simulink model "sfGetStartedBattery"  (R2025b)
settings: Solver=VariableStepAuto  StartTime=0.0  StopTime=inf  RelTol=1e-3
settings Model: Creator=The MathWorks, Inc.  LastModifiedBy=The MathWorks, Inc.

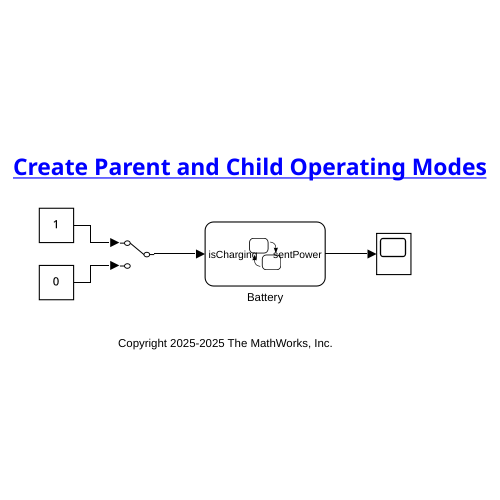
[thumbnail: Simulink's stored preview of the top-level diagram]
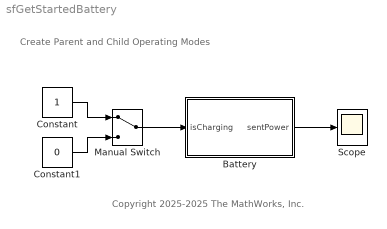
== system sfGetStartedBattery ==
  note: Copyright 2025-2025 The MathWorks, Inc.
  note: Create Parent and Child Operating Modes
  Battery : Stateflow chart  TreatAsAtomicUnit=on
  Constant : Constant
  Constant1 : Constant  Value=0
  Manual Switch : ManualSwitch
  Scope : Scope
      settings: ActiveDisplayYMinimum=-0.43749999999999989  ActiveDisplayYMaximum=3.9375
  wires:
  Manual Switch/1 -> Battery/1(isCharging)
  Constant/1 -> Manual Switch/1
  Constant1/1 -> Manual Switch/2
  Battery/1(sentPower) -> Scope/1

== stateflow chart sfGetStartedBattery/Battery ==
  state Charge
    entry:
    sentPower=0;
    during:
    charge=charge+4;
  state Discharge
    entry:
    sentPower=3.5;
    during:
    charge=charge-3;
  (default) -> Charge
  Charge -> Discharge : [~isCharging]
  Discharge -> Charge : [isCharging]
  data: isCharging input; sentPower output; charge local =50
